simulink model "MPSFP3NFGA"  (R2026b)
settings: Solver=ode15s  MaxStep=1E-3
libraries: slpidlib x1
settings Model: LastModifiedBy=Neltzon Farid
settings DataIOCC: DSMLogging=off  ReturnWorkspaceOutputs=off  SaveOutput=off  SignalLogging=off  TimeSaveName=t
settings DebuggingCC: AlgebraicLoopMsg=none  ArtificialAlgebraicLoopMsg=none  MaxConsecutiveZCsMsg=none
settings SimscapeCC: SimscapeLogType=all  SimscapeNominalValues="[{\"value\":\"1\",\"unit\":\"A\"},{\"value\":\"1\",\"unit\":\"bar\"},{\"value\":\"1\",\"unit\":\"cm^2\"},{\"value\":\"1\",\"unit\":\"cm^3/s\"},{\"value\":\"1\",\"unit\":\"kJ/kg\"},{\"value\":\"1\",\"unit\":\"kW\"},{\"value\":\"1\",\"unit\":\"l\"},{\"value\":\"1\",\"unit\":\"N\"},{\"value\":\"1\",\"unit\":\"N*m\"},{\"value\":\"1\",\"unit\":\"V\"},{\"value\":\"0.001\",\"unit\":\"Wb\"}]"  SimscapeUseEnergyAccounting=off

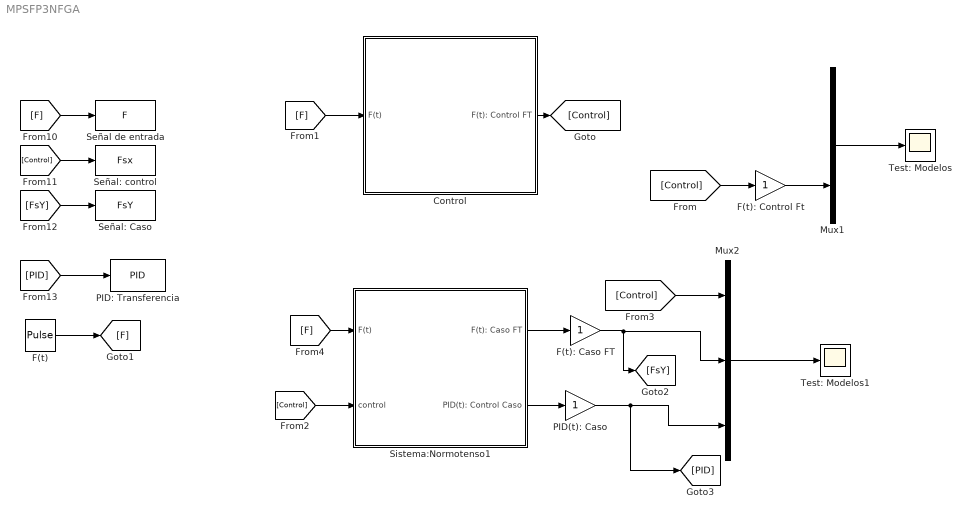
== system MPSFP3NFGA ==
  Control : Subsystem
  F(t) : DiscretePulseGenerator  PulseType=Time based  Period=10  PulseWidth=10  PhaseDelay=1
  F(t): Caso FT : Gain
  F(t): Control Ft : Gain
  Mux1 : Mux  Inputs=2
  Mux2 : Mux  Inputs=3
  PID(t): Caso : Gain
  PID: Transferencia : ToWorkspace  VariableName=PID  SampleTime=-1
  Señal de entrada : ToWorkspace  VariableName=F  SampleTime=-1
  Señal: Caso : ToWorkspace  VariableName=FsY  SampleTime=-1
  Señal: control : ToWorkspace  VariableName=Fsx  SampleTime=-1
  Sistema:Normotenso1 : Subsystem
  Test: Modelos : Scope
      settings: ActiveDisplayYMinimum=-0.74388631619415779  ActiveDisplayYMaximum=1.6755428307479283  YLabel=V(t)
  Test: Modelos1 : Scope
      settings: ActiveDisplayYMinimum=-0.74389  ActiveDisplayYMaximum=1.2755  YLabel=V(t)
  wires:
  Mux1/1 -> Test: Modelos/1
  [F] -> Control/1(F(t))
  [Control] -> Señal: control/1
  [FsY] -> Señal: Caso/1
  [F] -> Señal de entrada/1
  [PID] -> PID: Transferencia/1
  F(t)/1 -> [F]
  Control/1(F(t): Control FT) -> [Control]
  [Control] -> F(t): Control Ft/1
  F(t): Control Ft/1 -> Mux1/2
  Sistema:Normotenso1/2(PID(t): Control Caso) -> PID(t): Caso/1
  Mux2/1 -> Test: Modelos1/1
  [Control] -> Sistema:Normotenso1/2(control)
  [F] -> Sistema:Normotenso1/1(F(t))
  Sistema:Normotenso1/1(F(t): Caso FT) -> F(t): Caso FT/1
  F(t): Caso FT/1 -> Mux2/2, [FsY]
  [Control] -> Mux2/1
  PID(t): Caso/1 -> [PID], Mux2/3

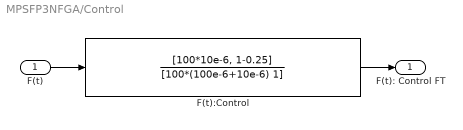
== system MPSFP3NFGA/Control ==
  F(t) : Inport
  F(t):Control : TransferFcn  Numerator=[100*10e-6, 1-0.25]  Denominator=[100*(100e-6+10e-6) 1]
  F(t): Control FT : Outport
  wires:
  F(t)/1 -> F(t):Control/1
  F(t):Control/1 -> F(t): Control FT/1

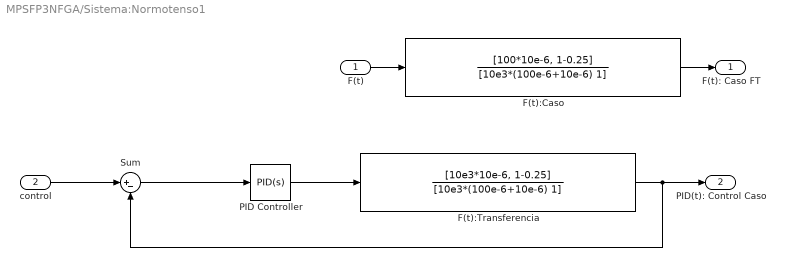
== system MPSFP3NFGA/Sistema:Normotenso1 ==
  F(t) : Inport
  control : Inport  Port=2
  F(t):Caso : TransferFcn  Numerator=[100*10e-6, 1-0.25]  Denominator=[10e3*(100e-6+10e-6) 1]
  F(t):Transferencia : TransferFcn  Numerator=[10e3*10e-6, 1-0.25]  Denominator=[10e3*(100e-6+10e-6) 1]
  PID Controller : slpidlib/PID Controller  Controller=PID  Form=Parallel  TimeDomain=Continuous-time  UseExternalTs=off  SampleTime=-1  IntegratorMethod=Forward Euler  FilterMethod=Forward Euler  ControllerParametersSource=internal  P=0.021474668154024  I=42258.7709415255  UseKiTs=off  D=0  UseExternalDerivativeSource=off  N=100  UseFilter=on  TunerSelectOption=Transfer Function Based (PID Tuner App)  InitialConditionSource=internal  InitialConditionForIntegrator=0  InitialConditionForFilter=0  DifferentiatorICPrevScaledInput=0  ExternalReset=none  TrackingMode=off  Kt=1  LimitOutput=off  SatLimitsSource=internal  UpperSaturationLimit=inf  LowerSaturationLimit=-inf  LinearizeAsGain=on  AntiWindupMode=none  Kb=1  LimitIntegrator=off  UpperIntegratorSaturationLimit=inf  LowerIntegratorSaturationLimit=-inf  POutMin=[]  POutMax=[]  IOutMin=[]  IOutMax=[]  DOutMin=[]  DOutMax=[]  NOutMin=[]  NOutMax=[]  SumOutMin=[]  SumOutMax=[]  SaturationOutMin=[]  SaturationOutMax=[]  PParamMin=[]  PParamMax=[]  IParamMin=[]  IParamMax=[]  DParamMin=[]  DParamMax=[]  NParamMin=[]  NParamMax=[]  KbParamMin=[]  KbParamMax=[]  KtParamMin=[]  KtParamMax=[]  KbOutMin=[]  KbOutMax=[]  KtOutMin=[]  KtOutMax=[]  IntegratorOutMin=[]  IntegratorOutMax=[]  FilterOutMin=[]  FilterOutMax=[]  SumI1OutMin=[]  SumI1OutMax=[]  SumI2OutMin=[]  SumI2OutMax=[]  SumI3OutMin=[]  SumI3OutMax=[]  SumI4OutMin=[]  SumI4OutMax=[]  SumDOutMin=[]  SumDOutMax=[]  DifferentiatorOutMin=[]  DifferentiatorOutMax=[]  FilterDiffOutCoefMin=[]  FilterDiffOutCoefMax=[]  ReciprocalOutMin=[]  ReciprocalOutMax=[]  SumDenOutMin=[]  SumDenOutMax=[]  SumNumOutMin=[]  SumNumOutMax=[]  DivideOutMin=[]  DivideOutMax=[]  UdiffTsProdOutMin=[]  UdiffTsProdOutMax=[]  NTsProdOutMin=[]  NTsProdOutMax=[]  UintegralTsProdOutMin=[]  UintegralTsProdOutMax=[]  UngainTsProdOutMin=[]  UngainTsProdOutMax=[]  ClampingZeroOutDataTypeStr=Inherit: Inherit via back propagation  ClampingZeroOutMin=[]  ClampingZeroOutMax=[]  FilterDenConstantOutDataTypeStr=Inherit: Inherit via back propagation  FilterDenConstantOutMin=[]  FilterDenConstantOutMax=[]  PCopyOutDataTypeStr=Inherit: Inherit via back propagation  PCopyOutMin=[]  PCopyOutMax=[]  NCopyOutDataTypeStr=Inherit: Inherit via back propagation  NCopyOutMin=[]  NCopyOutMax=[]  IntegratorContinuousStateAttributes=''  IntegratorStateMustResolveToSignalObject=off  IntegratorRTWStateStorageClass=Auto  FilterContinuousStateAttributes=''  FilterStateMustResolveToSignalObject=off  FilterRTWStateStorageClass=Auto  ParallelPVariant=InternalParameters  IdealPVariant=Disabled  IVariant=InternalParameters  DVariant=InternalParameters  IntegratorVariant=Continuous  SatVariant=Disabled  AWVariant=Passthrough  PCopyVariant=Disabled  TRVariant=Disabled  FdbkBlocksVariant=Forward  IdealPFdbkVariant=Disabled  SatFdbkVariant=Disabled  DerivativeFilterVariant=ContFilter  NVariant=InternalParameters  NCopyVariant=Disabled  FilterICVariant=InternalICsFilter  IntegratorICVariant=InternalICs  ExternalResetVariant=Disabled  TRSumVariant=Passthrough  SumFdbkVariant=Disabled  SumVariant=Sum_PID  TsampFilterVariant=InternalTs  TsampNgainVariant=Passthrough  TsampIntegralVariant=Disabled_SignalSpec  ExternalSaturationOutDataTypeStr=Inherit: Same as second input  DerivativeSourceVariant=ErrorSignal  PreIntVariant=InternalPreInt
  Sum : Sum  Inputs=|+-
  F(t): Caso FT : Outport
  PID(t): Control Caso : Outport  Port=2
  wires:
  F(t)/1 -> F(t):Caso/1
  F(t):Caso/1 -> F(t): Caso FT/1
  F(t):Transferencia/1 -> Sum/2, PID(t): Control Caso/1
  PID Controller/1 -> F(t):Transferencia/1
  Sum/1 -> PID Controller/1
  control/1 -> Sum/1
